simulink model "s_b4a4x32kf"  (R2018a)
settings: Solver=VariableStepDiscrete  StartTime=0.0  StopTime=1  RelTol=1e-3
undefined symbols (not defined in the file): fft_stages, n_bits_ants, n_bits_xengs
libraries: xbsIndex_r4 x22056, xbsReplacements_r4 x30, casper_library_misc x29, casper_library_scopes x15, xps_library x4
(part 62 of 227)

== system s_b4a4x32kf/sys0/vacc/status ==
  out_acc_cnt : Inport
  out_err_cnt : Inport  Port=2
  out_arm_cnt : Inport  Port=3
  out_ld_cnt : Inport  Port=4
  assert_acc_cnt : xbsIndex_r4/Assert  assert_type=on  type_source=Explicitly  gui_display_data_type=Fixed-point  arith_type=Unsigned  n_bits=12  bin_pt=0  preci_type=Single  exp_width=8  frac_width=24  assert_rate=off  rate_source=Explicitly  period=1  output_port=on  block_type=assert
  assert_arm_cnt : xbsIndex_r4/Assert  assert_type=on  type_source=Explicitly  gui_display_data_type=Fixed-point  arith_type=Unsigned  n_bits=4  bin_pt=0  preci_type=Single  exp_width=8  frac_width=24  assert_rate=off  rate_source=Explicitly  period=1  output_port=on  block_type=assert
  assert_err_cnt : xbsIndex_r4/Assert  assert_type=on  type_source=Explicitly  gui_display_data_type=Fixed-point  arith_type=Unsigned  n_bits=12  bin_pt=0  preci_type=Single  exp_width=8  frac_width=24  assert_rate=off  rate_source=Explicitly  period=1  output_port=on  block_type=assert
  assert_ld_cnt : xbsIndex_r4/Assert  assert_type=on  type_source=Explicitly  gui_display_data_type=Fixed-point  arith_type=Unsigned  n_bits=4  bin_pt=0  preci_type=Single  exp_width=8  frac_width=24  assert_rate=off  rate_source=Explicitly  period=1  output_port=on  block_type=assert
  cast_gw : xbsIndex_r4/Convert  gui_display_data_type=Fixed-point  arith_type=Unsigned  n_bits=32  bin_pt=0  float_type=Single  exp_bits=8  fraction_bits=24  quantization=Truncate  overflow=Wrap  en=off  latency=1  pipeline=off  dbl_ovrd=off  block_type=convert
  concatenate : xbsIndex_r4/Concat  num_inputs=4  dbl_ovrd=off  block_type=concat
  io_delay : xbsIndex_r4/Delay  rst=off  infoeditControl=Selection of Reset will increase slice count due to use of real FFs and instead of SRLs  en=off  latency=1  reg_retiming=on  dbl_ovrd=off  block_type=delay
  reint{1..4} (4 alike) : xbsIndex_r4/Reinterpret  force_arith_type=on  arith_type=Unsigned  force_bin_pt=on  bin_pt=0  block_type=reinterpret
  s_b4a4x32kf_sys0_vacc_status_user_data_in : xbsIndex_r4/Gateway Out  inherit_from_input=off  hdl_port=on  rows=1  columns=1  UseAsDAC=off  DACChannel='1'  interface=None  automatic_assignment=on  address_offset=hex2dec('00')  intf_name=''  intf_description=''  timing_constraint=None  locs_specified=off  LOCs={}  io_standard={}  block_type=gatewayout
  sim_out : Terminator
  wires:
  concatenate/1 -> io_delay/1
  io_delay/1 -> cast_gw/1
  cast_gw/1 -> s_b4a4x32kf_sys0_vacc_status_user_data_in/1
  s_b4a4x32kf_sys0_vacc_status_user_data_in/1 -> sim_out/1
  out_acc_cnt/1 -> assert_acc_cnt/1
  assert_acc_cnt/1 -> reint1/1
  reint1/1 -> concatenate/1
  out_err_cnt/1 -> assert_err_cnt/1
  assert_err_cnt/1 -> reint2/1
  reint2/1 -> concatenate/2
  out_arm_cnt/1 -> assert_arm_cnt/1
  assert_arm_cnt/1 -> reint3/1
  reint3/1 -> concatenate/3
  out_ld_cnt/1 -> assert_ld_cnt/1
  assert_ld_cnt/1 -> reint4/1
  reint4/1 -> concatenate/4

== system s_b4a4x32kf/sys0/vacc/timestamp ==
  out_vacc_timestamp : Inport
  assert_vacc_timestamp : xbsIndex_r4/Assert  assert_type=on  type_source=Explicitly  gui_display_data_type=Fixed-point  arith_type=Unsigned  n_bits=32  bin_pt=0  preci_type=Single  exp_width=8  frac_width=24  assert_rate=off  rate_source=Explicitly  period=1  output_port=on  block_type=assert
  cast_gw : xbsIndex_r4/Convert  gui_display_data_type=Fixed-point  arith_type=Unsigned  n_bits=32  bin_pt=0  float_type=Single  exp_bits=8  fraction_bits=24  quantization=Truncate  overflow=Wrap  en=off  latency=1  pipeline=off  dbl_ovrd=off  block_type=convert
  io_delay : xbsIndex_r4/Delay  rst=off  infoeditControl=Selection of Reset will increase slice count due to use of real FFs and instead of SRLs  en=off  latency=0  reg_retiming=on  dbl_ovrd=off  block_type=delay
  reint1 : xbsIndex_r4/Reinterpret  force_arith_type=on  arith_type=Unsigned  force_bin_pt=on  bin_pt=0  block_type=reinterpret
  s_b4a4x32kf_sys0_vacc_timestamp_user_data_in : xbsIndex_r4/Gateway Out  inherit_from_input=off  hdl_port=on  rows=1  columns=1  UseAsDAC=off  DACChannel='1'  interface=None  automatic_assignment=on  address_offset=hex2dec('00')  intf_name=''  intf_description=''  timing_constraint=None  locs_specified=off  LOCs={}  io_standard={}  block_type=gatewayout
  sim_out : Terminator
  wires:
  io_delay/1 -> cast_gw/1
  cast_gw/1 -> s_b4a4x32kf_sys0_vacc_timestamp_user_data_in/1
  s_b4a4x32kf_sys0_vacc_timestamp_user_data_in/1 -> sim_out/1
  out_vacc_timestamp/1 -> assert_vacc_timestamp/1
  assert_vacc_timestamp/1 -> reint1/1
  reint1/1 -> io_delay/1

== system s_b4a4x32kf/sys0/vacc/vacc_monitor1 ==
  cnt_rst : Inport
  new_acc : Inport  Port=2
  error : Inport  Port=3
  Delay1 : Subsystem  Tag=cmac_delinked  mask(pipeline){csp_latency=2}
      mask prompts: csp_latency "Latency"
      mask help:
      | An explicitly laid-out delay line to avoid mapping to SRL16s
      | for use in pipelining to help achieve timing closure.
      mask init:
      | pipeline_init(gcb,'latency',csp_latency);
      settings: AttributesFormatString=Latency = %<latency>
      mask Display:
      | port_label('input', 1, 'd');
      | port_label('output', 1, 'q');
      | disp(['Z^-', num2str(csp_latency)]);
  Delay121 : Subsystem  Tag=cmac_delinked  mask(pipeline){csp_latency=2}
      mask prompts: csp_latency "Latency"
      mask help:
      | An explicitly laid-out delay line to avoid mapping to SRL16s
      | for use in pipelining to help achieve timing closure.
      mask init:
      | pipeline_init(gcb,'latency',csp_latency);
      settings: AttributesFormatString=Latency = %<latency>
      mask Display:
      | port_label('input', 1, 'd');
      | port_label('output', 1, 'q');
      | disp(['Z^-', num2str(csp_latency)]);
  Delay2 : Subsystem  Tag=cmac_delinked  mask(pipeline){csp_latency=2}
      mask prompts: csp_latency "Latency"
      mask help:
      | An explicitly laid-out delay line to avoid mapping to SRL16s
      | for use in pipelining to help achieve timing closure.
      mask init:
      | pipeline_init(gcb,'latency',csp_latency);
      settings: AttributesFormatString=Latency = %<latency>
      mask Display:
      | port_label('input', 1, 'd');
      | port_label('output', 1, 'q');
      | disp(['Z^-', num2str(csp_latency)]);
  Delay25 : Subsystem  Tag=cmac_delinked  mask(pipeline){csp_latency=2}
      mask prompts: csp_latency "Latency"
      mask help:
      | An explicitly laid-out delay line to avoid mapping to SRL16s
      | for use in pipelining to help achieve timing closure.
      mask init:
      | pipeline_init(gcb,'latency',csp_latency);
      settings: AttributesFormatString=Latency = %<latency>
      mask Display:
      | port_label('input', 1, 'd');
      | port_label('output', 1, 'q');
      | disp(['Z^-', num2str(csp_latency)]);
  Delay3 : Subsystem  Tag=cmac_delinked  mask(pipeline){csp_latency=2}
      mask prompts: csp_latency "Latency"
      mask help:
      | An explicitly laid-out delay line to avoid mapping to SRL16s
      | for use in pipelining to help achieve timing closure.
      mask init:
      | pipeline_init(gcb,'latency',csp_latency);
      settings: AttributesFormatString=Latency = %<latency>
      mask Display:
      | port_label('input', 1, 'd');
      | port_label('output', 1, 'q');
      | disp(['Z^-', num2str(csp_latency)]);
  payload_cnt1 : xbsIndex_r4/Counter  cnt_type=Free Running  cnt_to=0  operation=Up  start_count=0  cnt_by_val=1  arith_type=Unsigned  n_bits=12  bin_pt=0  load_pin=off  rst=on  en=on  explicit_period=off  period=1  use_behavioral_HDL=on  implementation=Fabric  use_rpm=on  dbl_ovrd=off  block_type=counter
      settings: xl_area=[0, 0, 0, 0, 0, 0, 0]
  payload_cnt3 : xbsIndex_r4/Counter  cnt_type=Free Running  cnt_to=0  operation=Up  start_count=0  cnt_by_val=1  arith_type=Unsigned  n_bits=12  bin_pt=0  load_pin=off  rst=on  en=on  explicit_period=off  period=1  use_behavioral_HDL=on  implementation=Fabric  use_rpm=on  dbl_ovrd=off  block_type=counter
      settings: xl_area=[0, 0, 0, 0, 0, 0, 0]
  acc_cnt : Outport
  error_cnt : Outport  Port=2
  wires:
  Delay2/1(q) -> payload_cnt3/2
  payload_cnt3/1 -> Delay121/1(d)
  Delay1/1(q) -> payload_cnt1/2
  payload_cnt1/1 -> Delay25/1(d)
  cnt_rst/1 -> Delay3/1(d)
  new_acc/1 -> Delay2/1(d)
  Delay25/1(q) -> error_cnt/1
  error/1 -> Delay1/1(d)
  Delay121/1(q) -> acc_cnt/1
  Delay3/1(q) -> payload_cnt1/1, payload_cnt3/1

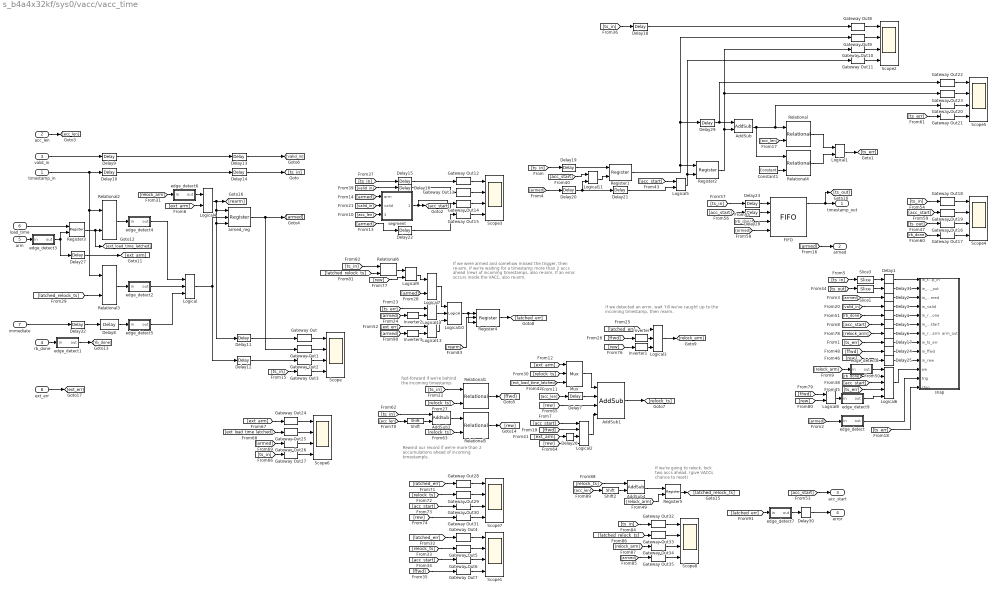
== system s_b4a4x32kf/sys0/vacc/vacc_time ==
  note: If we're going to relock,
      | lock two accs ahead.
      | (give VACCs chance to reset)
  note: If we were armed and somehow missed the
      | trigger, then re-arm.
      |
      | If we're waiting for a timestamp more than 2 accs ahead
      | (rew) of incoming timestamps, also re-arm.
      |
      | If an error occurs inside the VACC, also re-arm.
  note: If we detected an error,
      | wait 'till we've caught up to the incoming timestamp,
      | then rearm.
  note: fast-forward if we're
      | behind the incoming
      | timestamp.
  note: Rewind our record if we're more than
      | 2 accumulations ahead of incoming
      | timestampls.
  timestamp_in : Inport
  acc_len : Inport  Port=2
  valid_in : Inport  Port=3
  rb_done : Inport  Port=4
  arm : Inport  Port=5
  load_time : Inport  Port=6
  immediate : Inport  Port=7
  ext_err : Inport  Port=8
  AddSub : xbsIndex_r4/AddSub  mode=Subtraction  use_carryin=off  use_carryout=off  en=off  latency=1  precision=User Defined  arith_type=Unsigned  n_bits=timestamp_bits  bin_pt=0  quantization=Truncate  overflow=Wrap  use_behavioral_HDL=off  hw_selection=Fabric  pipelined=off  dbl_ovrd=off  block_type=addsub
  AddSub1 : xbsIndex_r4/AddSub  mode=Addition or Subtraction  use_carryin=off  use_carryout=off  en=on  latency=1  precision=User Defined  arith_type=Unsigned  n_bits=timestamp_bits  bin_pt=0  quantization=Truncate  overflow=Wrap  use_behavioral_HDL=on  hw_selection=Fabric  pipelined=off  dbl_ovrd=off  block_type=addsub
  AddSub2 : xbsIndex_r4/AddSub  mode=Addition  use_carryin=off  use_carryout=off  en=off  latency=1  precision=User Defined  arith_type=Unsigned  n_bits=timestamp_bits  bin_pt=0  quantization=Truncate  overflow=Wrap  use_behavioral_HDL=off  hw_selection=Fabric  pipelined=off  dbl_ovrd=off  block_type=addsub
  AddSub4 : xbsIndex_r4/AddSub  mode=Addition  use_carryin=off  use_carryout=off  en=off  latency=1  precision=User Defined  arith_type=Unsigned  n_bits=timestamp_bits  bin_pt=0  quantization=Truncate  overflow=Wrap  use_behavioral_HDL=off  hw_selection=Fabric  pipelined=off  dbl_ovrd=off  block_type=addsub
  Constant1 : xbsIndex_r4/Constant  const=0  gui_display_data_type=Fixed-point  arith_type=Unsigned  n_bits=1  bin_pt=0  preci_type=Single  exp_width=8  frac_width=24  explicit_period=on  period=1  equ=P=C  opselect=C  inp2=PCIN>>17  opr=+  inp1=P  carry=CIN  dbl_ovrd=off  block_type=constant
  Delay{1..6,17,24..25,31} (10 alike) : xbsIndex_r4/Delay  rst=off  infoeditControl=Selection of Reset will increase slice count due to use of real FFs and instead of SRLs  en=off  latency=4  reg_retiming=on  dbl_ovrd=off  block_type=delay
      Delay1 settings: infoedit=Hardware notes: A delay line is a chain, each link of which is an SRL16 or SRL32 followed by a flip-flop.
      Delay17 settings: infoedit=Hardware notes: A delay line is a chain, each link of which is an SRL16 or SRL32 followed by a flip-flop.
      Delay2 settings: infoedit=Hardware notes: A delay line is a chain, each link of which is an SRL16 or SRL32 followed by a flip-flop.
      Delay24 settings: infoedit=Hardware notes: A delay line is a chain, each link of which is an SRL16 or SRL32 followed by a flip-flop.
      Delay25 settings: infoedit=Hardware notes: A delay line is a chain, each link of which is an SRL16 or SRL32 followed by a flip-flop.
      Delay3 settings: infoedit=Hardware notes: A delay line is a chain, each link of which is an SRL16 or SRL32 followed by a flip-flop.
      Delay4 settings: infoedit=Hardware notes: A delay line is a chain, each link of which is an SRL16 or SRL32 followed by a flip-flop.
      Delay5 settings: infoedit=Hardware notes: A delay line is a chain, each link of which is an SRL16 or SRL32 followed by a flip-flop.
      Delay6 settings: infoedit=Hardware notes: A delay line is a chain, each link of which is an SRL16 or SRL32 followed by a flip-flop.
  Delay{7..14,23,26..29,32} (14 alike) : xbsIndex_r4/Delay  rst=off  infoeditControl=Selection of Reset will increase slice count due to use of real FFs and instead of SRLs  en=off  latency=1  reg_retiming=on  dbl_ovrd=off  block_type=delay
      Delay10 settings: infoedit=Hardware notes: A delay line is a chain, each link of which is an SRL16 or SRL32 followed by a flip-flop.
      Delay11 settings: infoedit=Hardware notes: A delay line is a chain, each link of which is an SRL16 or SRL32 followed by a flip-flop.
      Delay12 settings: infoedit=Hardware notes: A delay line is a chain, each link of which is an SRL16 or SRL32 followed by a flip-flop.
      Delay13 settings: infoedit=Hardware notes: A delay line is a chain, each link of which is an SRL16 or SRL32 followed by a flip-flop.
      Delay14 settings: infoedit=Hardware notes: A delay line is a chain, each link of which is an SRL16 or SRL32 followed by a flip-flop.
      Delay23 settings: infoedit=Hardware notes: A delay line is a chain, each link of which is an SRL16 or SRL32 followed by a flip-flop.
      Delay26 settings: infoedit=Hardware notes: A delay line is a chain, each link of which is an SRL16 or SRL32 followed by a flip-flop.
      Delay27 settings: infoedit=Hardware notes: A delay line is a chain, each link of which is an SRL16 or SRL32 followed by a flip-flop.
      Delay28 settings: infoedit=Hardware notes: A delay line is a chain, each link of which is an SRL16 or SRL32 followed by a flip-flop.
      Delay32 settings: infoedit=Hardware notes: A delay line is a chain, each link of which is an SRL16 or SRL32 followed by a flip-flop.
      Delay7 settings: infoedit=Hardware notes: A delay line is a chain, each link of which is an SRL16 or SRL32 followed by a flip-flop.
      Delay9 settings: infoedit=Hardware notes: A delay line is a chain, each link of which is an SRL16 or SRL32 followed by a flip-flop.
  Delay{15..16,18..22,30} (8 alike) : xbsIndex_r4/Delay  rst=off  infoeditControl=Selection of Reset will increase slice count due to use of real FFs and instead of SRLs  en=off  latency=2  reg_retiming=on  dbl_ovrd=off  block_type=delay
      settings: infoedit=Hardware notes: A delay line is a chain, each link of which is an SRL16 or SRL32 followed by a flip-flop.
  FIFO : xbsIndex_r4/FIFO  mem_type=Distributed RAM  performance_options=First_Word_Fall_Through  embedded_registers=off  depth=16  percent_nbits=1  rst=on  rst_latency=1  en=off  use_dcount=off  use_percent_full_port=off  use_almost_empty=off  almost_empty_thresh=2  use_almost_full=off  use_rd_rst_busy=off  use_wr_rst_busy=off  almost_full_thresh=14  explicit_period=off  dbl_ovrd=off  block_type=fifo
  Gateway Out{,1..35} (36 alike) : xbsIndex_r4/Gateway Out  inherit_from_input=off  hdl_port=on  rows=1  columns=1  UseAsDAC=off  DACChannel='1'  interface=None  automatic_assignment=on  address_offset=hex2dec('00')  intf_name=''  intf_description=''  timing_constraint=None  locs_specified=off  LOCs={}  io_standard={}  block_type=gatewayout
  Inverter{,1..3} (4 alike) : xbsIndex_r4/Inverter  en=off  latency=0  dbl_ovrd=off  block_type=inv
  Logical : xbsIndex_r4/Logical  logical_function=OR  inputs=3  en=off  latency=0  precision=Full  arith_type=Unsigned  n_bits=16  bin_pt=0  align_bp=on  dbl_ovrd=off  block_type=logical
  Logical{1,7,12..13} (4 alike) : xbsIndex_r4/Logical  logical_function=AND  inputs=2  en=off  latency=0  precision=Full  arith_type=Unsigned  n_bits=16  bin_pt=0  align_bp=on  dbl_ovrd=off  block_type=logical
  Logical10 : xbsIndex_r4/Logical  logical_function=OR  inputs=3  en=off  latency=0  precision=Full  arith_type=Unsigned  n_bits=16  bin_pt=0  align_bp=on  dbl_ovrd=off  block_type=logical
  Logical{4..5,8..9,11} (5 alike) : xbsIndex_r4/Logical  logical_function=OR  inputs=2  en=off  latency=0  precision=Full  arith_type=Unsigned  n_bits=16  bin_pt=0  align_bp=on  dbl_ovrd=off  block_type=logical
  Logical2 : xbsIndex_r4/Logical  logical_function=OR  inputs=4  en=off  latency=0  precision=Full  arith_type=Unsigned  n_bits=16  bin_pt=0  align_bp=on  dbl_ovrd=off  block_type=logical
  Logical3 : xbsIndex_r4/Logical  logical_function=AND  inputs=3  en=off  latency=0  precision=Full  arith_type=Unsigned  n_bits=16  bin_pt=0  align_bp=on  dbl_ovrd=off  block_type=logical
  Logical6 : xbsIndex_r4/Logical  logical_function=OR  inputs=5  en=off  latency=4  precision=Full  arith_type=Unsigned  n_bits=16  bin_pt=0  align_bp=on  dbl_ovrd=off  block_type=logical
  Mux : xbsIndex_r4/Mux  inputs=2  en=off  latency=1  precision=Full  arith_type=Unsigned  n_bits=16  bin_pt=14  quantization=Truncate  overflow=Wrap  dbl_ovrd=off  block_type=mux
  Register{1..3,5} (4 alike) : xbsIndex_r4/Register  init=0  rst=off  en=on  dbl_ovrd=off  block_type=register
  Register4 : xbsIndex_r4/Register  init=0  rst=on  en=on  dbl_ovrd=off  block_type=register
  Relational : xbsIndex_r4/Relational  mode=a!=b  op_type=Bool  en=off  latency=1  dbl_ovrd=off  block_type=relational
  Relational1 : xbsIndex_r4/Relational  mode=a>b  op_type=Bool  en=off  latency=1  dbl_ovrd=off  block_type=relational
  Relational2 : xbsIndex_r4/Relational  mode=a=b  op_type=Bool  en=off  latency=1  dbl_ovrd=off  block_type=relational
      settings: block_version=10.1.3
  Relational3 : xbsIndex_r4/Relational  mode=a=b  op_type=Bool  en=off  latency=1  dbl_ovrd=off  block_type=relational
      settings: block_version=10.1.3
  Relational4 : xbsIndex_r4/Relational  mode=a!=b  op_type=Bool  en=off  latency=1  dbl_ovrd=off  block_type=relational
  Relational5 : xbsIndex_r4/Relational  mode=a<b  op_type=Bool  en=off  latency=1  dbl_ovrd=off  block_type=relational
  Relational6 : xbsIndex_r4/Relational  mode=a>b  op_type=Bool  en=off  latency=1  dbl_ovrd=off  block_type=relational
  Scope{,1..8} (9 alike) : Scope  NumInputPorts=4
  Shift : xbsIndex_r4/Shift  shift_dir=Left  shift_bits=1  en=off  latency=0  precision=Full  arith_type="Signed  (2's comp)"  n_bits=16  bin_pt=14  quantization=Truncate  overflow=Wrap  dbl_ovrd=off  block_type=shift
  Shift2 : xbsIndex_r4/Shift  shift_dir=Left  shift_bits=1  en=off  latency=0  precision=Full  arith_type="Signed  (2's comp)"  n_bits=16  bin_pt=14  quantization=Truncate  overflow=Wrap  dbl_ovrd=off  block_type=shift
  Slice1 : xbsIndex_r4/Slice  nbits=24  boolean_output=off  mode=Lower Bit Location + Width  bit1=0  base1=MSB of Input  bit0=0  base0=LSB of Input  dbl_ovrd=off  block_type=slice
  Slice3 : xbsIndex_r4/Slice  nbits=24  boolean_output=off  mode=Lower Bit Location + Width  bit1=0  base1=MSB of Input  bit0=0  base0=LSB of Input  dbl_ovrd=off  block_type=slice
  armed_reg : xbsIndex_r4/Register  init=0  rst=on  en=on  dbl_ovrd=off  block_type=register
  edge_detect : Subsystem  mask(edge_detect){edge=Both, polarity=Active High, x_in=[0 0.08 0.08 0.16 0.16 0.24 0.24 0.32 0.32 0.4], y_in=[-1 -1  1  1  1  1  1  1  1  1], x_out=[0.6 0.68 0.68 0.76 0.76 0.84 0.84 0.92 0.92 1], y_out=[-1 -1  1  1 -1 -1 -1 -1 -1 -1]}
      mask prompts: edge "Edge Type"; polarity "Output Polarity"; x_in "Input X Positions"; y_in "Input Y Positions"; x_out "Output X Positions"; y_out "Output Y Positions"
      mask help: Output is active for one-cycle after each edge of the specified type (i.e. rising, falling or both).
      mask init: same as s_b4a4x32kf/edge_detect
      settings: AttributesFormatString=|
      | both edges
      | active high
      mask Help: Output is active for one-cycle after each edge of the specified type (i.e. rising, falling, or both).  Latency is zero.
      mask TypeOptions edge: Rising | Falling | Both
      mask TypeOptions polarity: Active High | Active Low
      mask Display:
      | plot(x_in_num,0.5+y_in_num*0.2);
      | plot(x_out_num,0.5+y_out_num*0.2);
  edge_detect1 : Subsystem  mask(edge_detect){edge=Rising, polarity=Active High, x_in=[0 0.08 0.08 0.16 0.16 0.24 0.24 0.32 0.32 0.4], y_in=[-1 -1  1  1  1  1  1  1  1  1], x_out=[0.6 0.68 0.68 0.76 0.76 0.84 0.84 0.92 0.92 1], y_out=[-1 -1  1  1 -1 -1 -1 -1 -1 -1]}
      mask prompts: edge "Edge Type"; polarity "Output Polarity"; x_in "Input X Positions"; y_in "Input Y Positions"; x_out "Output X Positions"; y_out "Output Y Positions"
      mask help: Output is active for one-cycle after each edge of the specified type (i.e. rising, falling or both).
      mask init: same as s_b4a4x32kf/edge_detect
      settings: AttributesFormatString=|
      | rising edges
      | active high
      mask Help: Output is active for one-cycle after each edge of the specified type (i.e. rising, falling, or both).  Latency is zero.
      mask TypeOptions edge: Rising | Falling | Both
      mask TypeOptions polarity: Active High | Active Low
      mask Display:
      | plot(x_in_num,0.5+y_in_num*0.2);
      | plot(x_out_num,0.5+y_out_num*0.2);
  edge_detect2 : Subsystem  mask(edge_detect){edge=Rising, polarity=Active High, x_in=[0 0.08 0.08 0.16 0.16 0.24 0.24 0.32 0.32 0.4], y_in=[-1 -1  1  1  1  1  1  1  1  1], x_out=[0.6 0.68 0.68 0.76 0.76 0.84 0.84 0.92 0.92 1], y_out=[-1 -1  1  1 -1 -1 -1 -1 -1 -1]}
      mask prompts: edge "Edge Type"; polarity "Output Polarity"; x_in "Input X Positions"; y_in "Input Y Positions"; x_out "Output X Positions"; y_out "Output Y Positions"
      mask help: Output is active for one-cycle after each edge of the specified type (i.e. rising, falling or both).
      mask init: same as s_b4a4x32kf/edge_detect
      settings: AttributesFormatString=|
      | rising edges
      | active high
      mask Help: Output is active for one-cycle after each edge of the specified type (i.e. rising, falling, or both).  Latency is zero.
      mask TypeOptions edge: Rising | Falling | Both
      mask TypeOptions polarity: Active High | Active Low
      mask Display:
      | plot(x_in_num,0.5+y_in_num*0.2);
      | plot(x_out_num,0.5+y_out_num*0.2);
  edge_detect3 : Subsystem  mask(edge_detect){edge=Rising, polarity=Active High, x_in=[0 0.08 0.08 0.16 0.16 0.24 0.24 0.32 0.32 0.4], y_in=[-1 -1  1  1  1  1  1  1  1  1], x_out=[0.6 0.68 0.68 0.76 0.76 0.84 0.84 0.92 0.92 1], y_out=[-1 -1  1  1 -1 -1 -1 -1 -1 -1]}
      mask prompts: edge "Edge Type"; polarity "Output Polarity"; x_in "Input X Positions"; y_in "Input Y Positions"; x_out "Output X Positions"; y_out "Output Y Positions"
      mask help: Output is active for one-cycle after each edge of the specified type (i.e. rising, falling or both).
      mask init: same as s_b4a4x32kf/edge_detect
      settings: AttributesFormatString=|
      | rising edges
      | active high
      mask Help: Output is active for one-cycle after each edge of the specified type (i.e. rising, falling, or both).  Latency is zero.
      mask TypeOptions edge: Rising | Falling | Both
      mask TypeOptions polarity: Active High | Active Low
      mask Display:
      | plot(x_in_num,0.5+y_in_num*0.2);
      | plot(x_out_num,0.5+y_out_num*0.2);
  edge_detect4 : Subsystem  mask(edge_detect){edge=Rising, polarity=Active High, x_in=[0 0.08 0.08 0.16 0.16 0.24 0.24 0.32 0.32 0.4], y_in=[-1 -1  1  1  1  1  1  1  1  1], x_out=[0.6 0.68 0.68 0.76 0.76 0.84 0.84 0.92 0.92 1], y_out=[-1 -1  1  1 -1 -1 -1 -1 -1 -1]}
      mask prompts: edge "Edge Type"; polarity "Output Polarity"; x_in "Input X Positions"; y_in "Input Y Positions"; x_out "Output X Positions"; y_out "Output Y Positions"
      mask help: Output is active for one-cycle after each edge of the specified type (i.e. rising, falling or both).
      mask init: same as s_b4a4x32kf/edge_detect
      settings: AttributesFormatString=|
      | rising edges
      | active high
      mask Help: Output is active for one-cycle after each edge of the specified type (i.e. rising, falling, or both).  Latency is zero.
      mask TypeOptions edge: Rising | Falling | Both
      mask TypeOptions polarity: Active High | Active Low
      mask Display:
      | plot(x_in_num,0.5+y_in_num*0.2);
      | plot(x_out_num,0.5+y_out_num*0.2);
  edge_detect5 : Subsystem  mask(edge_detect){edge=Rising, polarity=Active High, x_in=[0 0.08 0.08 0.16 0.16 0.24 0.24 0.32 0.32 0.4], y_in=[-1 -1  1  1  1  1  1  1  1  1], x_out=[0.6 0.68 0.68 0.76 0.76 0.84 0.84 0.92 0.92 1], y_out=[-1 -1  1  1 -1 -1 -1 -1 -1 -1]}
      mask prompts: edge "Edge Type"; polarity "Output Polarity"; x_in "Input X Positions"; y_in "Input Y Positions"; x_out "Output X Positions"; y_out "Output Y Positions"
      mask help: Output is active for one-cycle after each edge of the specified type (i.e. rising, falling or both).
      mask init: same as s_b4a4x32kf/edge_detect
      settings: AttributesFormatString=|
      | rising edges
      | active high
      mask Help: Output is active for one-cycle after each edge of the specified type (i.e. rising, falling, or both).  Latency is zero.
      mask TypeOptions edge: Rising | Falling | Both
      mask TypeOptions polarity: Active High | Active Low
      mask Display:
      | plot(x_in_num,0.5+y_in_num*0.2);
      | plot(x_out_num,0.5+y_out_num*0.2);
  edge_detect6 : Subsystem  mask(edge_detect){edge=Rising, polarity=Active High, x_in=[0 0.08 0.08 0.16 0.16 0.24 0.24 0.32 0.32 0.4], y_in=[-1 -1  1  1  1  1  1  1  1  1], x_out=[0.6 0.68 0.68 0.76 0.76 0.84 0.84 0.92 0.92 1], y_out=[-1 -1  1  1 -1 -1 -1 -1 -1 -1]}
      mask prompts: edge "Edge Type"; polarity "Output Polarity"; x_in "Input X Positions"; y_in "Input Y Positions"; x_out "Output X Positions"; y_out "Output Y Positions"
      mask help: Output is active for one-cycle after each edge of the specified type (i.e. rising, falling or both).
      mask init: same as s_b4a4x32kf/edge_detect
      settings: AttributesFormatString=|
      | rising edges
      | active high
      mask Help: Output is active for one-cycle after each edge of the specified type (i.e. rising, falling, or both).  Latency is zero.
      mask TypeOptions edge: Rising | Falling | Both
      mask TypeOptions polarity: Active High | Active Low
      mask Display:
      | plot(x_in_num,0.5+y_in_num*0.2);
      | plot(x_out_num,0.5+y_out_num*0.2);
  edge_detect7 : Subsystem  mask(edge_detect){edge=Both, polarity=Active High, x_in=[0 0.08 0.08 0.16 0.16 0.24 0.24 0.32 0.32 0.4], y_in=[-1 -1  1  1  1  1  1  1  1  1], x_out=[0.6 0.68 0.68 0.76 0.76 0.84 0.84 0.92 0.92 1], y_out=[-1 -1  1  1 -1 -1 -1 -1 -1 -1]}
      mask prompts: edge "Edge Type"; polarity "Output Polarity"; x_in "Input X Positions"; y_in "Input Y Positions"; x_out "Output X Positions"; y_out "Output Y Positions"
      mask help: Output is active for one-cycle after each edge of the specified type (i.e. rising, falling or both).
      mask init: same as s_b4a4x32kf/edge_detect
      settings: AttributesFormatString=|
      | both edges
      | active high
      mask Help: Output is active for one-cycle after each edge of the specified type (i.e. rising, falling, or both).  Latency is zero.
      mask TypeOptions edge: Rising | Falling | Both
      mask TypeOptions polarity: Active High | Active Low
      mask Display:
      | plot(x_in_num,0.5+y_in_num*0.2);
      | plot(x_out_num,0.5+y_out_num*0.2);
  edge_detect8 : Subsystem  mask(edge_detect){edge=Falling, polarity=Active High, x_in=[0 0.08 0.08 0.16 0.16 0.24 0.24 0.32 0.32 0.4], y_in=[-1 -1  1  1  1  1  1  1  1  1], x_out=[0.6 0.68 0.68 0.76 0.76 0.84 0.84 0.92 0.92 1], y_out=[-1 -1  1  1 -1 -1 -1 -1 -1 -1]}
      mask prompts: edge "Edge Type"; polarity "Output Polarity"; x_in "Input X Positions"; y_in "Input Y Positions"; x_out "Output X Positions"; y_out "Output Y Positions"
      mask help: Output is active for one-cycle after each edge of the specified type (i.e. rising, falling or both).
      mask init: same as s_b4a4x32kf/edge_detect
      settings: AttributesFormatString=|
      | falling edges
      | active high
      mask Help: Output is active for one-cycle after each edge of the specified type (i.e. rising, falling, or both).  Latency is zero.
      mask TypeOptions edge: Rising | Falling | Both
      mask TypeOptions polarity: Active High | Active Low
      mask Display:
      | plot(x_in_num,0.5+y_in_num*0.2);
      | plot(x_out_num,0.5+y_out_num*0.2);
  edge_detect9 : Subsystem  mask(edge_detect){edge=Both, polarity=Active High, x_in=[0 0.08 0.08 0.16 0.16 0.24 0.24 0.32 0.32 0.4], y_in=[-1 -1  1  1  1  1  1  1  1  1], x_out=[0.6 0.68 0.68 0.76 0.76 0.84 0.84 0.92 0.92 1], y_out=[-1 -1  1  1 -1 -1 -1 -1 -1 -1]}
      mask prompts: edge "Edge Type"; polarity "Output Polarity"; x_in "Input X Positions"; y_in "Input Y Positions"; x_out "Output X Positions"; y_out "Output Y Positions"
      mask help: Output is active for one-cycle after each edge of the specified type (i.e. rising, falling or both).
      mask init: same as s_b4a4x32kf/edge_detect
      settings: AttributesFormatString=|
      | both edges
      | active high
      mask Help: Output is active for one-cycle after each edge of the specified type (i.e. rising, falling, or both).  Latency is zero.
      mask TypeOptions edge: Rising | Falling | Both
      mask TypeOptions polarity: Active High | Active Low
      mask Display:
      | plot(x_in_num,0.5+y_in_num*0.2);
      | plot(x_out_num,0.5+y_out_num*0.2);
  segment : Subsystem
  snap : Subsystem  Tag=casper:bitsnap  AncestorBlock=casper_library_scopes/bitfield_snapshot  mask(bitsnap){io_names=[timestamp_in timestamp_out armed valid rb_done acc_start relock_arm ts_err ffwd rew], io_widths=[24 24 1 1 1 1 1 1 1 1], io_bps=0, io_types=[0 0 2 2 2 2 2 2 2 2], show_format=on, snap_storage=bram, snap_dram_dimm=2, snap_dram_clock=250, snap_nsamples=11, snap_data_width=64, snap_offset=off, snap_circap=on, snap_value=off, snap_ext_arm=off, snap_ext_circ=off, snap_provide_outputs=on, snap_use_dsp48=on, snap_delay=2, extra_names=[c d], extra_widths=[30 2], extra_bps=[0 0], extra_types=[0 0]}
      mask prompts: io_names "Names [msb...lsb]"; io_widths "Bitwidths [msb...lsb]"; io_bps "Binary pts [msb...lsb]"; io_types "Data types [msb...lsb], ufix=0, fix=1, bool=2"; show_format "Print format string?"; snap_storage "Storage medium"; snap_dram_dimm "DRAM dimm"; snap_dram_clock "DRAM clock rate"; snap_nsamples "Number of Samples (2^?)"; snap_data_width "Data width"; snap_offset "Start delay support"; snap_circap "Circular capture support"; snap_value "Extra value capture support"; snap_ext_arm "External arm support"; snap_ext_circ "External circular capture support"; snap_provide_outputs "Provide outputs"; snap_use_dsp48 "Use DSP48s to implement counters"; snap_delay "Pre-snapshot delay"; extra_names "Names [msb...lsb]"; extra_widths "Widths [msb...lsb]"; extra_bps "Binary pts [msb...lsb]"; extra_types "Data types [msb...lsb], ufix=0, fix=1, bool=2"
      mask help:
      | A wrapped snapshot block. Allows specification of inputs to a snapblock word so the toolflow can automatically set up the scope.
      | See documentation for snapshot for explanation of parameters.
      mask init:
      | bitsnap_init(gcb);
      settings: AttributesFormatString=|
      | snap(10):uf24.0,uf24.0,b,b,b,b,b,b,b,b = 56 bits\n64 wide, 2048 deep
      | debugID: 36008415
      mask TypeOptions snap_storage: bram | dram
      mask Callback snap_storage: bitsnap_callback();
      mask TypeOptions snap_dram_dimm: 1 | 2 | 3 | 4
      mask TypeOptions snap_dram_clock: 200 | 250 | 266 | 300 | 333
      mask TypeOptions snap_data_width: 8 | 16 | 32 | 64 | 128
      mask Callback snap_value: bitsnap_callback();
      mask Callback snap_ext_arm: bitsnap_callback();
      mask Callback snap_ext_circ: bitsnap_callback();
      mask Callback snap_provide_outputs: bitsnap_callback();
      mask DialogControl ParameterTabVar0 Prompt: Inputs
      mask DialogControl ParameterTabVar01 Prompt: Snapshot
      mask DialogControl ParameterTabVar012 Prompt: Extra Value
  timestamp_out : Outport
  armed : Outport  Port=2
  acc_start : Outport  Port=3
  error : Outport  Port=4
  wires:
  armed_reg/1 -> [armed], Gateway Out1/1
  rb_done/1 -> edge_detect1/1(in)
  Register2/1 -> Gateway Out23/1, Gateway Out10/1, AddSub/2
  AddSub/1 -> Gateway Out20/1, Relational/1, Relational4/1
  [acc_len] -> Relational/2
  Delay2/1 -> snap/3(in_armed)
  Delay3/1 -> snap/4(in_valid)
  Delay4/1 -> snap/5(in_rb_done)
  Logical6/1 -> snap/11(we)
  Delay7/1 -> AddSub1/2
  [armed] -> edge_detect/1(in)
  [armed] -> Delay2/1
  [armed] -> Delay20/1
  [ts_in] -> Slice3/1
  [acc_start] -> Delay5/1
  acc_len/1 -> [acc_len]
  [acc_len] -> segment/3(acc_len)
  [acc_len] -> Delay7/1
  Logical/1 -> armed_reg/2, Delay12/1
  arm/1 -> edge_detect3/1(in)
  load_time/1 -> Register3/1
  Register3/1 -> [ext_load_time_latched], Relational2/2
  immediate/1 -> Delay32/1
  Relational2/1 -> edge_detect4/1(in)
  Delay8/1 -> edge_detect5/1(in)
  Gateway Out/1 -> Scope/1
  Gateway Out1/1 -> Scope/2
  Gateway Out2/1 -> Scope/3
  Gateway Out3/1 -> Scope/4
  edge_detect4/1(out) -> Logical/1
  timestamp_in/1 -> Delay10/1, Relational3/1, Relational2/1
  [armed] -> segment/1(arm)
  Delay11/1 -> Gateway Out/1
  Delay12/1 -> Gateway Out2/1
  [ts_in] -> Gateway Out3/1
  [armed] -> armed/1
  [ts_err] -> snap/13(stop)
  [acc_start] -> Logical2/1
  Relational1/1 -> [ffwd]
  [ffwd] -> Logical2/2
  [valid_in] -> Delay3/1
  valid_in/1 -> Delay9/1
  [valid_in] -> segment/2(valid)
  Register4/1 -> [latched_err]
  [ffwd] -> Inverter/1
  [latched_err] -> Logical3/1
  Inverter/1 -> Logical3/2
  Relational3/1 -> edge_detect2/1(in)
  edge_detect2/1(out) -> Logical/2
  edge_detect5/1(out) -> Logical/3
  Logical4/1 -> [rearm], Delay11/1, armed_reg/3, armed_reg/1
  [ext_arm] -> Logical4/2
  [relock_arm] -> edge_detect6/1(in)
  edge_detect6/1(out) -> Logical4/1
  [relock_ts] -> Mux/2
  Mux/1 -> AddSub1/1
  [ext_load_time_latched] -> Mux/3
  Gateway Out4/1 -> Scope1/1
  Gateway Out5/1 -> Scope1/2
  Gateway Out6/1 -> Scope1/3
  Gateway Out7/1 -> Scope1/4
  [latched_err] -> Gateway Out4/1
  [relock_ts] -> Gateway Out5/1
  [acc_start] -> Gateway Out6/1
  [ffwd] -> Gateway Out7/1
  Gateway Out8/1 -> Scope2/1
  Gateway Out9/1 -> Scope2/2
  Gateway Out10/1 -> Scope2/3
  Gateway Out11/1 -> Scope2/4
  [ts_in] -> Delay18/1
  Inverter1/1 -> Logical3/3
  Logical11/1 -> Register1/2
  Delay9/1 -> Delay13/1
  Delay10/1 -> Delay14/1
  Delay13/1 -> [valid_in]
  Delay14/1 -> [ts_in]
  Gateway Out12/1 -> Scope3/1
  Gateway Out13/1 -> Scope3/2
  Gateway Out14/1 -> Scope3/3
  Gateway Out15/1 -> Scope3/4
  [ts_in] -> Delay15/1
  [valid_in] -> Delay16/1
  Delay15/1 -> Gateway Out12/1
  Delay16/1 -> Gateway Out13/1
  [armed] -> Delay22/1
  Delay18/1 -> Gateway Out8/1
  Delay19/1 -> Register1/1
  segment/1(acc_start) -> Gateway Out14/1, [acc_start]
  [ext_arm] -> Delay26/1
  [ext_arm] -> Mux/1
  Delay20/1 -> Logical11/2, Delay21/1
  Delay21/1 -> Logical5/2
  Logical5/1 -> Gateway Out11/1, Register2/2
  [acc_start] -> Logical5/1
  Delay22/1 -> Gateway Out15/1
  Gateway Out18/1 -> Scope4/1
  Gateway Out19/1 -> Scope4/2
  Gateway Out16/1 -> Scope4/3
  Gateway Out17/1 -> Scope4/4
  [acc_start] -> Logical11/1
  FIFO/1 -> [ts_out], timestamp_out/1
  edge_detect1/1(out) -> [rb_done]
  [ts_in] -> Delay19/1
  [ts_out] -> Gateway Out16/1
  [rb_done] -> Delay4/1
  edge_detect3/1(out) -> Register3/2, Delay27/1
  Slice3/1 -> Delay1/1
  [acc_start] -> acc_start/1
  [ts_in] -> Gateway Out18/1
  [rb_done] -> FIFO/3
  [acc_start] -> Delay28/1
  [ts_in] -> Delay23/1
  [armed] -> FIFO/4
  [acc_start] -> Gateway Out19/1
  [rb_done] -> Gateway Out17/1
  Delay23/1 -> FIFO/1
  Delay28/1 -> FIFO/2
  Gateway Out21/1 -> Scope5/4
  Gateway Out20/1 -> Scope5/3
  Gateway Out23/1 -> Scope5/2
  Gateway Out22/1 -> Scope5/1
  Constant1/1 -> Relational4/2
  Relational/1 -> Logical1/1
  Relational4/1 -> Logical1/2
  Logical1/1 -> [ts_err]
  [ts_err] -> Gateway Out21/1
  Register1/1 -> Register2/1, Delay29/1, Gateway Out9/1
  Delay29/1 -> Gateway Out22/1, AddSub/1
  Logical2/1 -> AddSub1/4
  Relational5/1 -> [rew]
  [rew] -> Logical2/4
  [rew] -> AddSub1/3
  [ts_in] -> Gateway Out27/1
  Gateway Out27/1 -> Scope6/4
  Gateway Out26/1 -> Scope6/3
  Gateway Out25/1 -> Scope6/2
  Gateway Out24/1 -> Scope6/1
  [ext_arm] -> Gateway Out24/1
  [ext_load_time_latched] -> Gateway Out25/1
  [armed] -> Gateway Out26/1
  [relock_ts] -> Relational5/2
  [ts_in] -> AddSub2/1
  AddSub2/1 -> Relational5/1
  [acc_len] -> Shift/1
  Shift/1 -> AddSub2/2
  [rew] -> Gateway Out31/1
  [acc_start] -> Gateway Out30/1
  [relock_ts] -> Gateway Out29/1
  [latched_err] -> Gateway Out28/1
  Gateway Out31/1 -> Scope7/4
  Gateway Out30/1 -> Scope7/3
  Gateway Out29/1 -> Scope7/2
  Gateway Out28/1 -> Scope7/1
  Delay30/1 -> error/1
  [rew] -> Inverter1/1
  Delay1/1 -> snap/1(in_timestamp_in)
  [ts_out] -> Slice1/1
  Slice1/1 -> Delay31/1
  Delay31/1 -> snap/2(in_timestamp_out)
  Delay5/1 -> snap/6(in_acc_start)
  [relock_arm] -> Delay6/1
  Delay6/1 -> snap/7(in_relock_arm)
  [rb_done] -> Logical6/2
  [acc_start] -> Logical6/3
  Delay17/1 -> snap/8(in_ts_err)
  [ts_err] -> Delay17/1
  [ts_err] -> Logical6/4
  Delay25/1 -> snap/10(in_rew)
  Delay24/1 -> snap/9(in_ffwd)
  [ffwd] -> Delay24/1
  [rew] -> Delay25/1
  edge_detect/1(out) -> snap/12(trig)
  [relock_arm] -> edge_detect8/1(in)
  edge_detect8/1(out) -> Logical6/1
  [ffwd] -> Logical8/1
  [rew] -> Logical8/2
  edge_detect9/1(out) -> Logical6/5
  Logical8/1 -> edge_detect9/1(in)
  [latched_relock_ts] -> Relational3/2
  Logical3/1 -> [relock_arm]
  Logical10/1 -> Register4/3, Register4/1
  [ts_err] -> Logical12/1
  [armed] -> Inverter2/1
  Inverter2/1 -> Logical12/2
  Logical12/1 -> Logical10/2
  [rearm] -> Register4/2
  Gateway Out35/1 -> Scope8/4
  Gateway Out34/1 -> Scope8/3
  Gateway Out33/1 -> Scope8/2
  Gateway Out32/1 -> Scope8/1
  [ts_in] -> Gateway Out32/1
  [armed] -> Gateway Out35/1
  [relock_ts] -> Relational1/2
  [ts_in] -> Relational1/1
  [latched_relock_ts] -> Relational6/2
  [ts_in] -> Relational6/1
  AddSub1/1 -> [relock_ts]
  [relock_arm] -> Register5/2
  Register5/1 -> [latched_relock_ts]
  [latched_relock_ts] -> Gateway Out33/1
  [relock_arm] -> Gateway Out34/1
  Shift2/1 -> AddSub4/2
  [relock_ts] -> AddSub4/1
  [acc_len] -> Shift2/1
  AddSub4/1 -> Register5/1
  Logical7/1 -> Logical10/1
  [armed] -> Logical7/2
  Relational6/1 -> Logical9/1
  Logical9/1 -> Logical7/1
  [rew] -> Logical9/2
  Delay26/1 -> Logical2/3
  Delay27/1 -> [ext_arm]
  Delay32/1 -> Delay8/1
  Inverter3/1 -> Logical13/2
  [armed] -> Inverter3/1
  [ext_err] -> Logical13/1
  Logical13/1 -> Logical10/3
  ext_err/1 -> [ext_err]
  [latched_err] -> edge_detect7/1(in)
  edge_detect7/1(out) -> Delay30/1

== system s_b4a4x32kf/sys0/vacc_tvg/bus_replicate1 ==
  in : Inport
  bussify : Subsystem  mask(bus_create){inputNum=8}
      mask prompts: inputNum "Number of inputs:"
      mask init:
      | bus_create_init(gcb,...
      |     'inputNum', inputNum);
  out : Outport
  wires:
  in/1 -> bussify/1(in1), bussify/2(in2), bussify/3(in3), bussify/4(in4), bussify/5(in5), bussify/6(in6), bussify/7(in7), bussify/8(in8)
  bussify/1(bus_out) -> out/1

== system s_b4a4x32kf/sys0/vacc_tvg/bus_replicate2 ==
  in : Inport
  bussify : Subsystem  mask(bus_create){inputNum=8}
      mask prompts: inputNum "Number of inputs:"
      mask init:
      | bus_create_init(gcb,...
      |     'inputNum', inputNum);
  out : Outport
  wires:
  in/1 -> bussify/1(in1), bussify/2(in2), bussify/3(in3), bussify/4(in4), bussify/5(in5), bussify/6(in6), bussify/7(in7), bussify/8(in8)
  bussify/1(bus_out) -> out/1

== system s_b4a4x32kf/sys0/vacc_tvg/edge_detect ==
  in : Inport
  Delay : xbsIndex_r4/Delay  rst=off  infoeditControl=Selection of Reset will increase slice count due to use of real FFs and instead of SRLs  en=off  latency=1  reg_retiming=off  dbl_ovrd=off  block_type=delay
      settings: xl_area=[0, 0, 0, 0, 0, 0, 0]
  Inverter : xbsIndex_r4/Inverter  en=off  latency=0  dbl_ovrd=off  block_type=inv
      settings: xl_area=[0, 0, 0, 0, 0, 0, 0]
  edge_op : xbsIndex_r4/Logical  logical_function=NOR  inputs=2  en=off  latency=0  precision=Full  arith_type=Unsigned  n_bits=8  bin_pt=2  align_bp=on  dbl_ovrd=off  block_type=logical
      settings: xl_area=[0, 0, 0, 0, 0, 0, 0]
  out : Outport
  wires:
  Delay/1 -> edge_op/2
  in/1 -> Delay/1, Inverter/1
  edge_op/1 -> out/1
  Inverter/1 -> edge_op/1

== system s_b4a4x32kf/sys0/vacc_tvg/edge_detect4 ==
  in : Inport
  Delay : xbsIndex_r4/Delay  rst=off  infoeditControl=Selection of Reset will increase slice count due to use of real FFs and instead of SRLs  en=off  latency=1  reg_retiming=on  dbl_ovrd=off  block_type=delay
      settings: xl_area=[0, 0, 0, 0, 0, 0, 0]
  Inverter : xbsIndex_r4/Inverter  en=off  latency=0  dbl_ovrd=off  block_type=inv
      settings: xl_area=[0, 0, 0, 0, 0, 0, 0]
  edge_op : xbsIndex_r4/Logical  logical_function=NOR  inputs=2  en=off  latency=0  precision=Full  arith_type=Unsigned  n_bits=8  bin_pt=2  align_bp=on  dbl_ovrd=off  block_type=logical
      settings: xl_area=[0, 0, 0, 0, 0, 0, 0]
  out : Outport
  wires:
  Inverter/1 -> edge_op/1
  edge_op/1 -> out/1
  in/1 -> Inverter/1, Delay/1
  Delay/1 -> edge_op/2

== system s_b4a4x32kf/sys0/vacc_tvg/generate_pulses ==
  run : Inport
  num_pulses : Inport  Port=2
  num_per_group : Inport  Port=3
  group period : Inport  Port=4
  Constant : xbsIndex_r4/Constant  const=777777  gui_display_data_type=Fixed-point  arith_type=Unsigned  n_bits=20  bin_pt=0  preci_type=Single  exp_width=8  frac_width=24  explicit_period=on  period=1  equ=P=C  opselect=C  inp2=PCIN>>17  opr=+  inp1=P  carry=CIN  dbl_ovrd=off  block_type=constant
  Gateway Out{1..8} (8 alike) : xbsIndex_r4/Gateway Out  inherit_from_input=off  hdl_port=off  rows=1  columns=1  UseAsDAC=off  DACChannel='1'  interface=None  automatic_assignment=on  address_offset=hex2dec('00')  intf_name=''  intf_description=''  timing_constraint=None  locs_specified=off  LOCs={}  io_standard={}  block_type=gatewayout
      settings: infoedit="Gateway out block.  Converts Xilinx fixed point inputs into ouputs of type Simulink integer, double, or fixed point.<P><P>Hardware notes:  In hardware these blocks become top level output ports or are discarded, depending on how they are configured."  xl_area=[0, 0, 0, 0, 0, 0, 0]  block_version=10.1.3
  Inverter : xbsIndex_r4/Inverter  en=off  latency=0  dbl_ovrd=off  block_type=inv
  Logical1 : xbsIndex_r4/Logical  logical_function=AND  inputs=2  en=off  latency=0  precision=Full  arith_type=Unsigned  n_bits=8  bin_pt=2  align_bp=on  dbl_ovrd=off  block_type=logical
      settings: xl_area=[0, 0, 0, 0, 0, 0, 0]
  Logical2 : xbsIndex_r4/Logical  logical_function=AND  inputs=3  en=off  latency=0  precision=Full  arith_type=Unsigned  n_bits=8  bin_pt=2  align_bp=on  dbl_ovrd=off  block_type=logical
      settings: xl_area=[0, 0, 0, 0, 0, 0, 0]
  Logical3 : xbsIndex_r4/Logical  logical_function=AND  inputs=3  en=off  latency=0  precision=Full  arith_type=Unsigned  n_bits=8  bin_pt=2  align_bp=on  dbl_ovrd=off  block_type=logical
      settings: xl_area=[0, 0, 0, 0, 0, 0, 0]
  Logical4 : xbsIndex_r4/Logical  logical_function=OR  inputs=2  en=off  latency=0  precision=Full  arith_type=Unsigned  n_bits=8  bin_pt=2  align_bp=off  dbl_ovrd=off  block_type=logical
      settings: xl_area=[0, 0, 0, 0, 0, 0, 0]
  Logical5 : xbsIndex_r4/Logical  logical_function=OR  inputs=2  en=off  latency=0  precision=Full  arith_type=Unsigned  n_bits=8  bin_pt=2  align_bp=on  dbl_ovrd=off  block_type=logical
      settings: xl_area=[0, 0, 0, 0, 0, 0, 0]
  Logical6 : xbsIndex_r4/Logical  logical_function=AND  inputs=2  en=off  latency=0  precision=Full  arith_type=Unsigned  n_bits=8  bin_pt=2  align_bp=on  dbl_ovrd=off  block_type=logical
      settings: xl_area=[0, 0, 0, 0, 0, 0, 0]
  Relational : xbsIndex_r4/Relational  mode=a>=b  op_type=Bool  en=off  latency=0  dbl_ovrd=off  block_type=relational
      settings: xl_area=[0, 0, 0, 0, 0, 0, 0]  block_version=10.1.3
  Relational1 : xbsIndex_r4/Relational  mode=a=b  op_type=Bool  en=off  latency=0  dbl_ovrd=off  block_type=relational
      settings: xl_area=[0, 0, 0, 0, 0, 0, 0]  block_version=10.1.3
  Relational2 : xbsIndex_r4/Relational  mode=a>b  op_type=Bool  en=off  latency=0  dbl_ovrd=off  block_type=relational
      settings: xl_area=[0, 0, 0, 0, 0, 0, 0]  block_version=10.1.3
  Relational3 : xbsIndex_r4/Relational  mode=a=b  op_type=Bool  en=off  latency=0  dbl_ovrd=off  block_type=relational
      settings: xl_area=[0, 0, 0, 0, 0, 0, 0]  block_version=10.1.3
  Scope1 : Scope  NumInputPorts=4
  Scope2 : Scope  NumInputPorts=4
  edge_detect : Subsystem  mask(edge_detect){edge=Rising, polarity=Active High, x_in=[0 0.08 0.08 0.16 0.16 0.24 0.24 0.32 0.32 0.4], y_in=[-1 -1  1  1  1  1  1  1  1  1], x_out=[0.6 0.68 0.68 0.76 0.76 0.84 0.84 0.92 0.92 1], y_out=[-1 -1  1  1 -1 -1 -1 -1 -1 -1]}
      mask prompts: edge "Edge Type"; polarity "Output Polarity"; x_in "Input X Positions"; y_in "Input Y Positions"; x_out "Output X Positions"; y_out "Output Y Positions"
      mask help: Output is active for one-cycle after each edge of the specified type (i.e. rising, falling or both).
      mask init: same as s_b4a4x32kf/edge_detect
      settings: AttributesFormatString=|
      | rising edges
      | active high
      mask Help: Output is active for one-cycle after each edge of the specified type (i.e. rising, falling, or both).  Latency is zero.
      mask TypeOptions edge: Rising | Falling | Both
      mask TypeOptions polarity: Active High | Active Low
      mask Display:
      | plot(x_in_num,0.5+y_in_num*0.2);
      | plot(x_out_num,0.5+y_out_num*0.2);
  group_cntr : xbsIndex_r4/Counter  cnt_type=Free Running  cnt_to=1  operation=Up  start_count=1  cnt_by_val=1  arith_type=Unsigned  n_bits=32  bin_pt=0  load_pin=off  rst=on  en=off  explicit_period=on  period=1  use_behavioral_HDL=off  implementation=Fabric  use_rpm=on  dbl_ovrd=off  block_type=counter
      settings: xl_area=[0, 0, 0, 0, 0, 0, 0]
  pulse_cntr : xbsIndex_r4/Counter  cnt_type=Free Running  cnt_to=1  operation=Up  start_count=0  cnt_by_val=1  arith_type=Unsigned  n_bits=32  bin_pt=0  load_pin=off  rst=on  en=on  explicit_period=on  period=1  use_behavioral_HDL=off  implementation=Fabric  use_rpm=on  dbl_ovrd=off  block_type=counter
      settings: xl_area=[0, 0, 0, 0, 0, 0, 0]
  tot_cntr : xbsIndex_r4/Counter  cnt_type=Free Running  cnt_to=1  operation=Up  start_count=1  cnt_by_val=1  arith_type=Unsigned  n_bits=32  bin_pt=0  load_pin=off  rst=on  en=on  explicit_period=on  period=1  use_behavioral_HDL=off  implementation=Fabric  use_rpm=on  dbl_ovrd=off  block_type=counter
      settings: xl_area=[0, 0, 0, 0, 0, 0, 0]
  valid : Outport
  running : Outport  Port=2
  wires:
  tot_cntr/1 -> Relational/2, Gateway Out1/1
  run/1 -> Logical3/3, Logical2/1, Gateway Out8/1, edge_detect/1(in)
  Logical5/1 -> running/1, Logical2/3, Logical3/1, Gateway Out2/1, Logical1/2
  num_pulses/1 -> Relational/1, Relational3/1
  edge_detect/1(out) -> tot_cntr/1, Gateway Out3/1, Logical4/1
  group_cntr/1 -> Relational1/2, Gateway Out5/1
  Relational1/1 -> Logical4/2
  pulse_cntr/1 -> Relational2/2, Gateway Out4/1
  Relational2/1 -> Logical2/2
  num_per_group/1 -> Relational2/1
  Logical2/1 -> Gateway Out7/1, Logical6/1, pulse_cntr/2
  Logical4/1 -> Inverter/1, pulse_cntr/1, group_cntr/1
  group period/1 -> Relational1/1
  Gateway Out5/1 -> Scope2/3
  Gateway Out4/1 -> Scope2/2
  Gateway Out6/1 -> Scope2/1
  Gateway Out1/1 -> Scope2/4
  Gateway Out7/1 -> Scope1/3
  Gateway Out3/1 -> Scope1/2
  Gateway Out8/1 -> Scope1/1
  Gateway Out2/1 -> Scope1/4
  Logical6/1 -> Logical3/2, Logical1/1
  Logical1/1 -> Gateway Out6/1, valid/1
  Logical3/1 -> tot_cntr/2
  Constant/1 -> Relational3/2
  Relational/1 -> Logical5/1
  Relational3/1 -> Logical5/2
  Inverter/1 -> Logical6/2
